simulink model "Series_winding_with_RL_load"  (R2025b)
settings: Solver=VariableStepAuto  StartTime=0.0  StopTime=0.1  FixedStep=1e-6  MaxStep=1e-6  RelTol=1e-4
values from neighbouring files (symbols this model uses):
  bias_current = 5    [parameters_for_AMB_topology.m]
  half_SW_Ts = SW_Ts*0.5    (= 2.5e-05)    [parameters_for_AMB_topology.m]
  K_i = 2*pi*f_c*R_value/U_dc    (= 47.1238898038)    [parameters_for_AMB_topology.m]
  K_p = 2*pi*f_c*L_value/U_dc    (= 0.0235619449019)    [parameters_for_AMB_topology.m]
  R_value = 1    [parameters_for_AMB_topology.m]
  SW_Ts = 1/(SW_frequency)    (= 5e-05)    [parameters_for_AMB_topology.m]
libraries: fl_lib x57, simulink x41, nesl_utility x33, eeGeneralControl x32, ee_lib x23
(part 5 of 5)

== system Series_winding_with_RL_load/PI_ctrl/Ictrl_anti_windup ==
  err : Inport
  AND : Logic  IconShape=distinctive  AllPortsSameDT=off  OutDataTypeStr=boolean
  Compare To Constant : simulink/Logic and Bit Operations/Compare To Constant  relop=<=  const=-1  OutDataTypeStr=boolean
  Compare To Constant1 : simulink/Logic and Bit Operations/Compare To Constant  relop=>=  const=1  OutDataTypeStr=boolean
  Compare To Constant2 : simulink/Logic and Bit Operations/Compare To Constant  relop=>=  const=0  OutDataTypeStr=boolean
  Constant : Constant  Value=0
  Gain1 : Gain  Gain=K_i
  Integrator : Integrator  LimitOutput=on  UpperSaturationLimit=1  LowerSaturationLimit=-1
  OR : Logic  Operator=OR  IconShape=distinctive  AllPortsSameDT=off  OutDataTypeStr=boolean
  Product : Product
  Switch : Switch  Criteria=u2 ~= 0  SaturateOnIntegerOverflow=off  InputSameDT=off
  Int_out : Outport
  wires:
  Compare To Constant2/1 -> AND/2
  Product/1 -> Compare To Constant2/1
  AND/1 -> Switch/2
  Constant/1 -> Switch/1
  Compare To Constant1/1 -> OR/2
  Switch/1 -> Gain1/1
  Gain1/1 -> Integrator/1
  Integrator/1 -> Int_out/1, Product/1, Compare To Constant1/1, Compare To Constant/1
  OR/1 -> AND/1
  Compare To Constant/1 -> OR/1
  err/1 -> Product/2, Switch/3

== system Series_winding_with_RL_load/PI_ctrl1/Ictrl_anti_windup ==
  err : Inport
  AND : Logic  IconShape=distinctive  AllPortsSameDT=off  OutDataTypeStr=boolean
  Compare To Constant : simulink/Logic and Bit Operations/Compare To Constant  relop=<=  const=-1  OutDataTypeStr=boolean
  Compare To Constant1 : simulink/Logic and Bit Operations/Compare To Constant  relop=>=  const=1  OutDataTypeStr=boolean
  Compare To Constant2 : simulink/Logic and Bit Operations/Compare To Constant  relop=>=  const=0  OutDataTypeStr=boolean
  Constant : Constant  Value=0
  Gain1 : Gain  Gain=K_i
  Integrator : Integrator  LimitOutput=on  UpperSaturationLimit=1  LowerSaturationLimit=-1
  OR : Logic  Operator=OR  IconShape=distinctive  AllPortsSameDT=off  OutDataTypeStr=boolean
  Product : Product
  Switch : Switch  Criteria=u2 ~= 0  SaturateOnIntegerOverflow=off  InputSameDT=off
  Int_out : Outport
  wires:
  Compare To Constant2/1 -> AND/2
  Product/1 -> Compare To Constant2/1
  AND/1 -> Switch/2
  Constant/1 -> Switch/1
  Compare To Constant1/1 -> OR/2
  Switch/1 -> Gain1/1
  Gain1/1 -> Integrator/1
  Integrator/1 -> Int_out/1, Product/1, Compare To Constant1/1, Compare To Constant/1
  OR/1 -> AND/1
  Compare To Constant/1 -> OR/1
  err/1 -> Product/2, Switch/3

== system Series_winding_with_RL_load/PI_ctrl2/Ictrl_anti_windup ==
  err : Inport
  AND : Logic  IconShape=distinctive  AllPortsSameDT=off  OutDataTypeStr=boolean
  Compare To Constant : simulink/Logic and Bit Operations/Compare To Constant  relop=<=  const=-1  OutDataTypeStr=boolean
  Compare To Constant1 : simulink/Logic and Bit Operations/Compare To Constant  relop=>=  const=1  OutDataTypeStr=boolean
  Compare To Constant2 : simulink/Logic and Bit Operations/Compare To Constant  relop=>=  const=0  OutDataTypeStr=boolean
  Constant : Constant  Value=0
  Gain1 : Gain  Gain=K_i
  Integrator : Integrator  LimitOutput=on  UpperSaturationLimit=1  LowerSaturationLimit=-1
  OR : Logic  Operator=OR  IconShape=distinctive  AllPortsSameDT=off  OutDataTypeStr=boolean
  Product : Product
  Switch : Switch  Criteria=u2 ~= 0  SaturateOnIntegerOverflow=off  InputSameDT=off
  Int_out : Outport
  wires:
  Compare To Constant2/1 -> AND/2
  Product/1 -> Compare To Constant2/1
  AND/1 -> Switch/2
  Constant/1 -> Switch/1
  Compare To Constant1/1 -> OR/2
  Switch/1 -> Gain1/1
  Gain1/1 -> Integrator/1
  Integrator/1 -> Int_out/1, Product/1, Compare To Constant1/1, Compare To Constant/1
  OR/1 -> AND/1
  Compare To Constant/1 -> OR/1
  err/1 -> Product/2, Switch/3

== system Series_winding_with_RL_load/PI_ctrl3/Ictrl_anti_windup ==
  err : Inport
  AND : Logic  IconShape=distinctive  AllPortsSameDT=off  OutDataTypeStr=boolean
  Compare To Constant : simulink/Logic and Bit Operations/Compare To Constant  relop=<=  const=-1  OutDataTypeStr=boolean
  Compare To Constant1 : simulink/Logic and Bit Operations/Compare To Constant  relop=>=  const=1  OutDataTypeStr=boolean
  Compare To Constant2 : simulink/Logic and Bit Operations/Compare To Constant  relop=>=  const=0  OutDataTypeStr=boolean
  Constant : Constant  Value=0
  Gain1 : Gain  Gain=K_i
  Integrator : Integrator  LimitOutput=on  UpperSaturationLimit=1  LowerSaturationLimit=-1
  OR : Logic  Operator=OR  IconShape=distinctive  AllPortsSameDT=off  OutDataTypeStr=boolean
  Product : Product
  Switch : Switch  Criteria=u2 ~= 0  SaturateOnIntegerOverflow=off  InputSameDT=off
  Int_out : Outport
  wires:
  Compare To Constant2/1 -> AND/2
  Product/1 -> Compare To Constant2/1
  AND/1 -> Switch/2
  Constant/1 -> Switch/1
  Compare To Constant1/1 -> OR/2
  Switch/1 -> Gain1/1
  Gain1/1 -> Integrator/1
  Integrator/1 -> Int_out/1, Product/1, Compare To Constant1/1, Compare To Constant/1
  OR/1 -> AND/1
  Compare To Constant/1 -> OR/1
  err/1 -> Product/2, Switch/3

== system Series_winding_with_RL_load/PI_ctrl4/Ictrl_anti_windup ==
  err : Inport
  AND : Logic  IconShape=distinctive  AllPortsSameDT=off  OutDataTypeStr=boolean
  Compare To Constant : simulink/Logic and Bit Operations/Compare To Constant  relop=<=  const=-1  OutDataTypeStr=boolean
  Compare To Constant1 : simulink/Logic and Bit Operations/Compare To Constant  relop=>=  const=1  OutDataTypeStr=boolean
  Compare To Constant2 : simulink/Logic and Bit Operations/Compare To Constant  relop=>=  const=0  OutDataTypeStr=boolean
  Constant : Constant  Value=0
  Gain1 : Gain  Gain=K_i
  Integrator : Integrator  LimitOutput=on  UpperSaturationLimit=1  LowerSaturationLimit=-1
  OR : Logic  Operator=OR  IconShape=distinctive  AllPortsSameDT=off  OutDataTypeStr=boolean
  Product : Product
  Switch : Switch  Criteria=u2 ~= 0  SaturateOnIntegerOverflow=off  InputSameDT=off
  Int_out : Outport
  wires:
  Compare To Constant2/1 -> AND/2
  Product/1 -> Compare To Constant2/1
  AND/1 -> Switch/2
  Constant/1 -> Switch/1
  Compare To Constant1/1 -> OR/2
  Switch/1 -> Gain1/1
  Gain1/1 -> Integrator/1
  Integrator/1 -> Int_out/1, Product/1, Compare To Constant1/1, Compare To Constant/1
  OR/1 -> AND/1
  Compare To Constant/1 -> OR/1
  err/1 -> Product/2, Switch/3

== system Series_winding_with_RL_load/PI_ctrl5/Ictrl_anti_windup ==
  err : Inport
  AND : Logic  IconShape=distinctive  AllPortsSameDT=off  OutDataTypeStr=boolean
  Compare To Constant : simulink/Logic and Bit Operations/Compare To Constant  relop=<=  const=-1  OutDataTypeStr=boolean
  Compare To Constant1 : simulink/Logic and Bit Operations/Compare To Constant  relop=>=  const=1  OutDataTypeStr=boolean
  Compare To Constant2 : simulink/Logic and Bit Operations/Compare To Constant  relop=>=  const=0  OutDataTypeStr=boolean
  Constant : Constant  Value=0
  Gain1 : Gain  Gain=K_i
  Integrator : Integrator  LimitOutput=on  UpperSaturationLimit=1  LowerSaturationLimit=-1
  OR : Logic  Operator=OR  IconShape=distinctive  AllPortsSameDT=off  OutDataTypeStr=boolean
  Product : Product
  Switch : Switch  Criteria=u2 ~= 0  SaturateOnIntegerOverflow=off  InputSameDT=off
  Int_out : Outport
  wires:
  Compare To Constant2/1 -> AND/2
  Product/1 -> Compare To Constant2/1
  AND/1 -> Switch/2
  Constant/1 -> Switch/1
  Compare To Constant1/1 -> OR/2
  Switch/1 -> Gain1/1
  Gain1/1 -> Integrator/1
  Integrator/1 -> Int_out/1, Product/1, Compare To Constant1/1, Compare To Constant/1
  OR/1 -> AND/1
  Compare To Constant/1 -> OR/1
  err/1 -> Product/2, Switch/3

== system Series_winding_with_RL_load/PI_ctrl6/Ictrl_anti_windup ==
  err : Inport
  AND : Logic  IconShape=distinctive  AllPortsSameDT=off  OutDataTypeStr=boolean
  Compare To Constant : simulink/Logic and Bit Operations/Compare To Constant  relop=<=  const=-1  OutDataTypeStr=boolean
  Compare To Constant1 : simulink/Logic and Bit Operations/Compare To Constant  relop=>=  const=1  OutDataTypeStr=boolean
  Compare To Constant2 : simulink/Logic and Bit Operations/Compare To Constant  relop=>=  const=0  OutDataTypeStr=boolean
  Constant : Constant  Value=0
  Gain1 : Gain  Gain=K_i
  Integrator : Integrator  LimitOutput=on  UpperSaturationLimit=1  LowerSaturationLimit=-1
  OR : Logic  Operator=OR  IconShape=distinctive  AllPortsSameDT=off  OutDataTypeStr=boolean
  Product : Product
  Switch : Switch  Criteria=u2 ~= 0  SaturateOnIntegerOverflow=off  InputSameDT=off
  Int_out : Outport
  wires:
  Compare To Constant2/1 -> AND/2
  Product/1 -> Compare To Constant2/1
  AND/1 -> Switch/2
  Constant/1 -> Switch/1
  Compare To Constant1/1 -> OR/2
  Switch/1 -> Gain1/1
  Gain1/1 -> Integrator/1
  Integrator/1 -> Int_out/1, Product/1, Compare To Constant1/1, Compare To Constant/1
  OR/1 -> AND/1
  Compare To Constant/1 -> OR/1
  err/1 -> Product/2, Switch/3

== system Series_winding_with_RL_load/PI_ctrl7/Ictrl_anti_windup ==
  err : Inport
  AND : Logic  IconShape=distinctive  AllPortsSameDT=off  OutDataTypeStr=boolean
  Compare To Constant : simulink/Logic and Bit Operations/Compare To Constant  relop=<=  const=-1  OutDataTypeStr=boolean
  Compare To Constant1 : simulink/Logic and Bit Operations/Compare To Constant  relop=>=  const=1  OutDataTypeStr=boolean
  Compare To Constant2 : simulink/Logic and Bit Operations/Compare To Constant  relop=>=  const=0  OutDataTypeStr=boolean
  Constant : Constant  Value=0
  Gain1 : Gain  Gain=K_i
  Integrator : Integrator  LimitOutput=on  UpperSaturationLimit=1  LowerSaturationLimit=-1
  OR : Logic  Operator=OR  IconShape=distinctive  AllPortsSameDT=off  OutDataTypeStr=boolean
  Product : Product
  Switch : Switch  Criteria=u2 ~= 0  SaturateOnIntegerOverflow=off  InputSameDT=off
  Int_out : Outport
  wires:
  Compare To Constant2/1 -> AND/2
  Product/1 -> Compare To Constant2/1
  AND/1 -> Switch/2
  Constant/1 -> Switch/1
  Compare To Constant1/1 -> OR/2
  Switch/1 -> Gain1/1
  Gain1/1 -> Integrator/1
  Integrator/1 -> Int_out/1, Product/1, Compare To Constant1/1, Compare To Constant/1
  OR/1 -> AND/1
  Compare To Constant/1 -> OR/1
  err/1 -> Product/2, Switch/3

== system Series_winding_with_RL_load/PI_ctrl8/Ictrl_anti_windup ==
  err : Inport
  AND : Logic  IconShape=distinctive  AllPortsSameDT=off  OutDataTypeStr=boolean
  Compare To Constant : simulink/Logic and Bit Operations/Compare To Constant  relop=<=  const=-1  OutDataTypeStr=boolean
  Compare To Constant1 : simulink/Logic and Bit Operations/Compare To Constant  relop=>=  const=1  OutDataTypeStr=boolean
  Compare To Constant2 : simulink/Logic and Bit Operations/Compare To Constant  relop=>=  const=0  OutDataTypeStr=boolean
  Constant : Constant  Value=0
  Gain1 : Gain  Gain=K_i
  Integrator : Integrator  LimitOutput=on  UpperSaturationLimit=1  LowerSaturationLimit=-1
  OR : Logic  Operator=OR  IconShape=distinctive  AllPortsSameDT=off  OutDataTypeStr=boolean
  Product : Product
  Switch : Switch  Criteria=u2 ~= 0  SaturateOnIntegerOverflow=off  InputSameDT=off
  Int_out : Outport
  wires:
  Compare To Constant2/1 -> AND/2
  Product/1 -> Compare To Constant2/1
  AND/1 -> Switch/2
  Constant/1 -> Switch/1
  Compare To Constant1/1 -> OR/2
  Switch/1 -> Gain1/1
  Gain1/1 -> Integrator/1
  Integrator/1 -> Int_out/1, Product/1, Compare To Constant1/1, Compare To Constant/1
  OR/1 -> AND/1
  Compare To Constant/1 -> OR/1
  err/1 -> Product/2, Switch/3

== system Series_winding_with_RL_load/PI_ctrl9/Ictrl_anti_windup ==
  err : Inport
  AND : Logic  IconShape=distinctive  AllPortsSameDT=off  OutDataTypeStr=boolean
  Compare To Constant : simulink/Logic and Bit Operations/Compare To Constant  relop=<=  const=-1  OutDataTypeStr=boolean
  Compare To Constant1 : simulink/Logic and Bit Operations/Compare To Constant  relop=>=  const=1  OutDataTypeStr=boolean
  Compare To Constant2 : simulink/Logic and Bit Operations/Compare To Constant  relop=>=  const=0  OutDataTypeStr=boolean
  Constant : Constant  Value=0
  Gain1 : Gain  Gain=K_i
  Integrator : Integrator  LimitOutput=on  UpperSaturationLimit=1  LowerSaturationLimit=-1
  OR : Logic  Operator=OR  IconShape=distinctive  AllPortsSameDT=off  OutDataTypeStr=boolean
  Product : Product
  Switch : Switch  Criteria=u2 ~= 0  SaturateOnIntegerOverflow=off  InputSameDT=off
  Int_out : Outport
  wires:
  Compare To Constant2/1 -> AND/2
  Product/1 -> Compare To Constant2/1
  AND/1 -> Switch/2
  Constant/1 -> Switch/1
  Compare To Constant1/1 -> OR/2
  Switch/1 -> Gain1/1
  Gain1/1 -> Integrator/1
  Integrator/1 -> Int_out/1, Product/1, Compare To Constant1/1, Compare To Constant/1
  OR/1 -> AND/1
  Compare To Constant/1 -> OR/1
  err/1 -> Product/2, Switch/3

== matlab function Series_winding_with_RL_load/MATLAB Function ==
  data: u input; cmin output; cmax output
function [cmin, cmax] = minmax(u)

c_sorted = sort(u);      % 升序
cmin = c_sorted(1);      % 首 = 最小
cmax = c_sorted(end);    % 末 = 最大



end
